simulink model "MPPT_HITL_Test"  (R2024a)
settings: Solver=FixedStepAuto  StartTime=0.0  StopTime=inf  RelTol=1e-3
libraries: c2837xDlib x3, c2802xlib x2
settings Model: Creator=k_boumbi  LastModifiedBy=k_boumbi

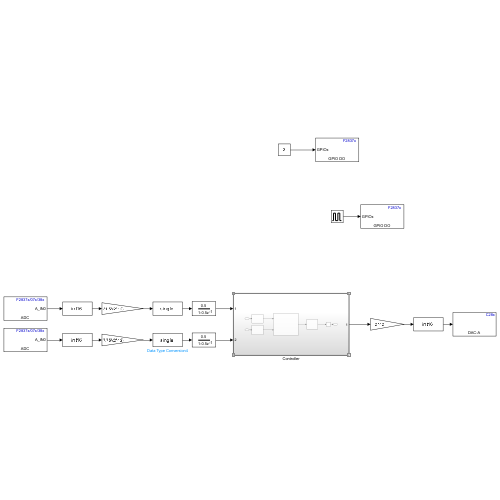
[thumbnail: Simulink's stored preview of the top-level diagram]
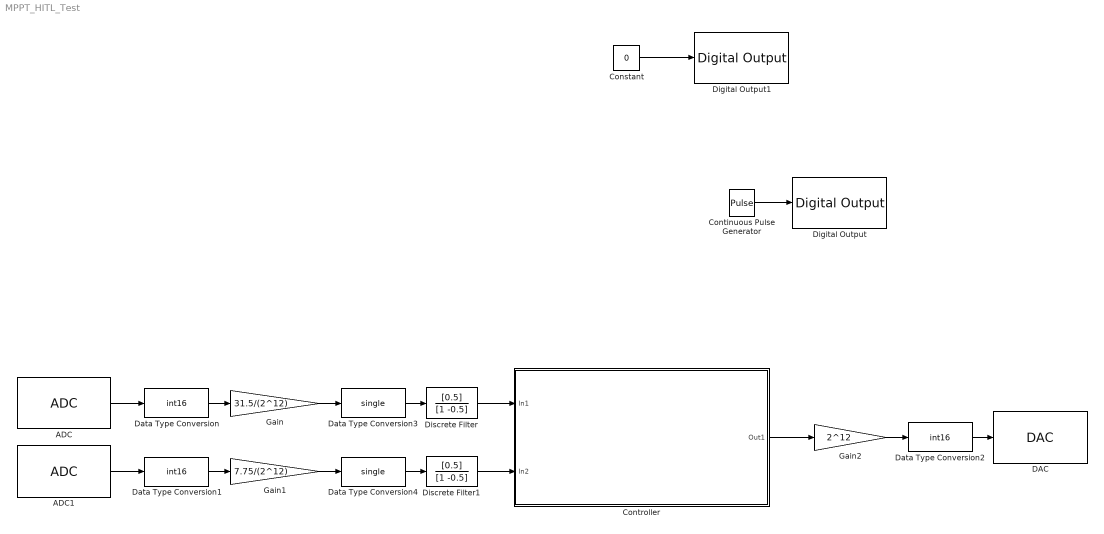
== system MPPT_HITL_Test ==
  ADC : c2802xlib/ADC  blkParamProc=C2000_Type4  ADCModule=A  samplingMode=Single sample mode  ADCResolution=12-bit (Single-ended input)  useSOC1=SOC0  useSOC2=SOC0_SOC1  SOCAcquisitionWindow=15  SOCTriggerSource=Software  SOCInterruptTrigger=No ADCINT  Ts=0.001  dType=uint16  postInterrupt=off  interruptSel=ADCINT1  ADCINTContinuous=on  endma=off  chdma=1  conv1=ADCINA0  conv2=ADCINA0 and ADCINB0  conv1_Type4=ADCIN0  conv2_Type4=ADCIN0 and ADCIN1
      settings: LibrarySourceBlock=c2837xDlib/ADC
  ADC1 : c2802xlib/ADC  blkParamProc=C2000_Type4  ADCModule=A  samplingMode=Single sample mode  ADCResolution=12-bit (Single-ended input)  useSOC1=SOC0  useSOC2=SOC0_SOC1  SOCAcquisitionWindow=15  SOCTriggerSource=Software  SOCInterruptTrigger=No ADCINT  Ts=0.001  dType=uint16  postInterrupt=off  interruptSel=ADCINT1  ADCINTContinuous=on  endma=off  chdma=1  conv1=ADCINA0  conv2=ADCINA0 and ADCINB0  conv1_Type4=ADCIN0  conv2_Type4=ADCIN0 and ADCIN1
      settings: LibrarySourceBlock=c2837xDlib/ADC
  Constant : Constant  Value=0
  Continuous Pulse Generator : DiscretePulseGenerator  PulseType=Time based  Period=1  PulseWidth=50
  Controller : Subsystem
  DAC : c2837xDlib/DAC  channel=A  saturate=off
  Data Type Conversion : DataTypeConversion  OutDataTypeStr=int16  SaturateOnIntegerOverflow=off  RndMeth=Floor
  Data Type Conversion1 : DataTypeConversion  OutDataTypeStr=int16  SaturateOnIntegerOverflow=off  RndMeth=Floor
  Data Type Conversion2 : DataTypeConversion  OutDataTypeStr=int16  SaturateOnIntegerOverflow=off  RndMeth=Floor
  Data Type Conversion3 : DataTypeConversion  OutDataTypeStr=single  SaturateOnIntegerOverflow=off  RndMeth=Floor
  Data Type Conversion4 : DataTypeConversion  OutDataTypeStr=single  SaturateOnIntegerOverflow=off  RndMeth=Floor
  Digital Output : c2837xDlib/Digital Output  GPIO_Number=GPIO0~GPIO7  GPIO_Bit0=on  GPIO_BIT0_Toggle=off  GPIO_Bit1=off  GPIO_BIT1_Toggle=off  GPIO_Bit2=off  GPIO_BIT2_Toggle=off  GPIO_Bit3=off  GPIO_BIT3_Toggle=off  GPIO_Bit4=off  GPIO_BIT4_Toggle=off  GPIO_Bit5=off  GPIO_BIT5_Toggle=off  GPIO_Bit6=off  GPIO_BIT6_Toggle=off  GPIO_Bit7=off  GPIO_BIT7_Toggle=off
  Digital Output1 : c2837xDlib/Digital Output  GPIO_Number=GPIO0~GPIO7  GPIO_Bit0=on  GPIO_BIT0_Toggle=off  GPIO_Bit1=off  GPIO_BIT1_Toggle=off  GPIO_Bit2=off  GPIO_BIT2_Toggle=off  GPIO_Bit3=off  GPIO_BIT3_Toggle=off  GPIO_Bit4=off  GPIO_BIT4_Toggle=off  GPIO_Bit5=off  GPIO_BIT5_Toggle=off  GPIO_Bit6=off  GPIO_BIT6_Toggle=off  GPIO_Bit7=off  GPIO_BIT7_Toggle=off
  Discrete Filter : DiscreteFilter  Numerator=[0.5]  Denominator=[1 -0.5]
  Discrete Filter1 : DiscreteFilter  Numerator=[0.5]  Denominator=[1 -0.5]
  Gain : Gain  Gain=31.5/(2^12)
  Gain1 : Gain  Gain=7.75/(2^12)
  Gain2 : Gain  Gain=2^12
  wires:
  Constant/1 -> Digital Output1/1
  Data Type Conversion2/1 -> DAC/1
  Gain2/1 -> Data Type Conversion2/1
  Data Type Conversion1/1 -> Gain1/1
  ADC1/1 -> Data Type Conversion1/1
  Data Type Conversion/1 -> Gain/1
  ADC/1 -> Data Type Conversion/1
  Data Type Conversion3/1 -> Discrete Filter/1
  Data Type Conversion4/1 -> Discrete Filter1/1
  Gain/1 -> Data Type Conversion3/1
  Gain1/1 -> Data Type Conversion4/1
  Discrete Filter1/1 -> Controller/2(In2)
  Discrete Filter/1 -> Controller/1(In1)
  Controller/1(Out1) -> Gain2/1
  Continuous Pulse Generator/1 -> Digital Output/1

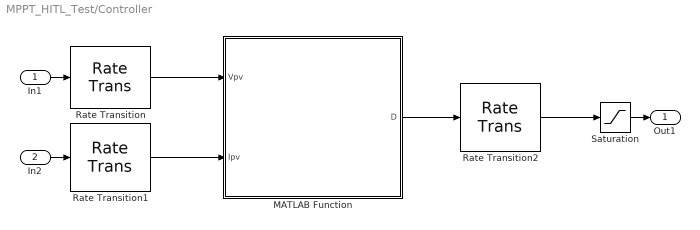
== system MPPT_HITL_Test/Controller ==
  In1 : Inport
  In2 : Inport  Port=2
  MATLAB Function : MATLAB Function  InitFcn=params  TreatAsAtomicUnit=on
  Rate Transition : RateTransition
  Rate Transition1 : RateTransition
  Rate Transition2 : RateTransition
  Saturation : Saturate
  Out1 : Outport
  wires:
  Rate Transition1/1 -> MATLAB Function/2(Ipv)
  In1/1 -> Rate Transition/1
  Rate Transition/1 -> MATLAB Function/1(Vpv)
  Rate Transition2/1 -> Saturation/1
  MATLAB Function/1(D) -> Rate Transition2/1
  In2/1 -> Rate Transition1/1
  Saturation/1 -> Out1/1

== matlab function MPPT_HITL_Test/Controller/MATLAB Function ==
  data: Vpv input; D output; Ipv input
function D = MPPT_PO_C2000(Vpv, Ipv)
%MPPT_PO_C2000  Perturb & Observe MPPT, written for code generation on the
%   TI F28379D (single precision, persistent state, no dynamic memory).
%
%   Inputs : Vpv [V], Ipv [A]  (already scaled and filtered, type single)
%   Output : D   duty-cycle command in [D_MIN, D_MAX]
%
%   Sign convention: for a buck or boost with the battery on the output,
%   increasing D LOWERS the PV voltage. If your topology does the opposite,
%   swap the "+" and "-" on the duty-cycle update below.
%
%   Run this block at the slow MPPT rate (e.g. 10-100 Hz), not at the ADC
%   rate, so the converter settles between perturbations.

% ---- Tuning parameters ----
D_STEP = single(0.005);   % perturbation size
D_MIN  = single(0.05);    % keep away from 0 and 1
D_MAX  = single(0.95);
D_INIT = single(0.5);
P_DEADBAND = single(0.2); % [W] ignore power changes smaller than this (noise)

% ---- State kept between calls ----
persistent Dk Vprev Pprev
if isempty(Dk)
    Dk    = D_INIT;
    Vprev = single(0);
    Pprev = single(0);
end

% ---- P&O step ----
P  = Vpv * Ipv;
dP = P   - Pprev;
dV = Vpv - Vprev;

if abs(dP) > P_DEADBAND
    if (dP > 0) == (dV > 0)
        % Power rose while voltage rose (or fell while voltage fell):
        % the MPP is at a higher voltage -> raise Vpv -> lower D
        Dk = Dk - D_STEP;
    else
        % The MPP is at a lower voltage -> lower Vpv -> raise D
        Dk = Dk + D_STEP;
    end
end

% Clamp the duty cycle
Dk = min(max(Dk, D_MIN), D_MAX);

Vprev = Vpv;
Pprev = P;
D = Dk;
end
